simulink library "mssSimulink"  (R2024a)
settings: Solver=ode45  StartTime=0.0  StopTime=10.0  RelTol=1e-3
undefined symbols (not defined in the file): ABC, CN_data, CX_data, CY_data, D, G, Hoerner, K_supply, kt2ms, MA, magnitude, MRB, pathlength, RAO_Amp, RAO_Dir, RAO_Freq, RAO_Phase, RAO_Vel, RAO_yaw_back, RAO_yaw_quant, RAO_yaw_quantization_flag, rho_a, slcm, T_supply, table, vessel, vesselABC
libraries: $bdroot x99, simulink x13
(part 2 of 9)

== system mssSimulink/Marine craft models ==
  note: 3-DOF low-speed models
  note: 6-DOF low-speed models 6-DOF interface for 3-DOF models
  note: m-file models
  note: 4-DOF maneuveing models
  note: Nomoto models
  4-DOF naval vessel : Subsystem  mask(Naval Vessel Nonlinear Manoeuvring Model){x0=[kt2ms(15),0,0,0,0,0]'}
      mask prompts: x0 "Initial Condition x0=[u,v,p,r,phi,psi]"
      mask help:
      | Naval Vessel Model in 4 DOFs (surge,sway, roll, and yaw)
      | Input:
      | tau - vector of forces [X,Y,K,N]' in Newtons
      |
      | Output:
      | eta -  [phi,psi]'  Euler angles [rad]
      | nu  -  [u,v,p,r]   Linear and angular velocities in the body-fixed frame.
      |
      | Copyright 2005 NTNU
      | Author: Tristan Perez
      mask Help:
      | <p><font face="Arial">This is nonlinear manoeuvring model in 4 DOFs. This model
      | has been implemented usign the GNC vessel model block, and the </font>
      | <font face="Courier">m</font><font face="Arial"> file associated with the model
      | is </font></p>
      | <p><font face="Courier">MSS\VESSELS\navalvessel.m</font></p>
      | <p><font face="Arial">All the hydrodynamic data is in the above file.&nbsp; For
      | an example of use see&nbsp; the following demo:</font></p>
      | <p><font face="Courier">SIMULINK\DEMOS\demoNavalVesselMano.slxl</font></p>
      mask Display:
      | image(imread('simulink/figs/nvessel.jpg'))
      | color('white'); port_label('output', 1, 'eta')
      | color('white');port_label('output', 2, 'nu')
      | color('white'); port_label('input', 1, 'tau')
  6-DOF semisub : Subsystem  InitFcn=load MSS/VESSELS/models/rigModel/rig.mat  mask(6-DOF semisub){D=D, G=G, MA=MA, MRB=MRB}
      mask prompts: D "Linear damping matrix: D"; G "Spring matrix G:"; MA "System inertia added mass matrix: M"; MRB "System inertia rigid-body matrix"
      mask help:
      | Semisub low-speed model for DP.
      |
      | Inputs:
      |
      |    tau = 6 DOF control input vector (generalized force)
      |
      | Outputs:
      |
      |    eta = [x, y, z, phi, theta, psi]'
      |    nu  = [u, v, w, p, q, r]'
      mask Display:
      | image(imread('semisub.jpg'))
      | color('black'); port_label('output', 1, 'eta')
      | color('black'); port_label('output', 2, 'nu')
      | color('black'); port_label('input', 1, 'tau')
      | color('black'); port_label('input', 2, 'nu_c')
  6-DOF supply vessel interface : Subsystem
      mask Display: disp('6-DOF interface\n to 3-DOF vessel\n models')
  Container ship: L = 175 m : Subsystem  mask(m-file vessel model interface){vessmodel='container', dimu_model=2, dimx_model=10}
      mask prompts: vessmodel "m-file vessel model"; dimu_model "dim u"; dimx_model "dim x"
      mask help:
      | Simulink interface to the GNC toolbox m-file vessel models, type:
      |
      |    >help vesselmodels
      |
      | in the Matlab command window. A Simulink demo file is found under examples (demomf.mdl).
      |
      | Inputs/outputs:
      |
      |    u   = control input vector of dimension dimu
      |    xo = initial state vector of dimension dimx
      |    x   = state vector of dimension dimx
      mask Help:
      | Simulink interface to the GNC toolbox m-file vessel models.
      | Type >help vesselmodels in the Matlab command window to see a list of the m-file vessel models. The dimension of the state and input vectors are found  by typing >help "m-file"
      mask Display: disp('Integration of\n container.m\n\n x = [u v r x y psi p phi delta n]\n u = [delta_c n_c]')
  CyberShipII : Subsystem  LoadFcn=initCS2
      mask init:
      | D = [ 2.0000         0         0
      |          0    7.0000    0.1000
      |          0    0.1000    0.5000];
      | M = [  25.8000         0         0
      |          0   33.8000    1.0115
      |          0    1.0115    2.7600 ];
      mask Display:
      | image(imread('simulink/figs/cs.jpg'))
      | color('white'); port_label('output', 1, 'eta')
      | color('white');port_label('output', 2, 'nu')
      | color('white'); port_label('input', 1, 'tau')
  Deep submergence rescue vehicle (DSRV.m) : Subsystem
      mask Display: image('DSRV.jpg'); % Use "Edit Image" on toolstrip to change.
  Large tanker: L = 304 m : Subsystem  mask(m-file vessel model interface){vessmodel='tanker', dimu_model=3, dimx_model=8}
      mask prompts: vessmodel "m-file vessel model"; dimu_model "dim u"; dimx_model "dim x"
      mask help:
      | Simulink interface to the GNC toolbox m-file vessel models, type:
      |
      |    >help vesselmodels
      |
      | in the Matlab command window. A Simulink demo file is found under examples (demomf.mdl).
      |
      | Inputs/outputs:
      |
      |    u   = control input vector of dimension dimu
      |    xo = initial state vector of dimension dimx
      |    x   = state vector of dimension dimx
      mask Help:
      | Simulink interface to the GNC toolbox m-file vessel models.
      | Type >help vesselmodels in the Matlab command window to see a list of the m-file vessel models. The dimension of the state and input vectors are found  by typing >help "m-file"
      mask Display: disp('Integration of\n tanker.m\n\n x = [u v r x y psi delta n]\n u = [delta_c n_c h]')
  Mariner class cargo ship (2nd -order) : Subsystem  mask(Container ship (2nd-order model)){rate_max=5*(pi/180), delta_max=20*(pi/180), K=0.185, T1=118, T2=7.8, T3=18.5}
      mask prompts: rate_max "Max rudder rate: rate_max (rad/s)"; delta_max "Max rudder angle: delta_max (rad)"; K "Gain constant: K (1/s)"; T1 "Time constant: T1 (s)"; T2 "Time constant: T2 (s)"; T3 "Time constant: T3 (s)"
      mask Display:
      | image(imread('simulink/figs/mariner.jpg'))
      | color('white'); port_label('output', 1, 'psi')
      | color('white'); port_label('output', 2, 'r')
      | color('white'); port_label('output', 3, 'delta')
      | color('white'); port_label('input', 1, 'delta_c')
  Mariner class cargo ship (mariner.m) : Subsystem
      mask Display: image('mariner.jpg');
  Naval Postgraduate School AUV (npsAUV.m) : Subsystem
      mask Display: image('npsauv.png'); % Use "Edit Image" on toolstrip to change.
  Otter USV (otter.m) : Subsystem
      mask Display: image('otter.jpg'); % Use "Edit Image" on toolstrip to change.
  Remus 100 AUV (remus100.m) : Subsystem
      mask Display: image('remus100.jpg'); % Use "Edit Image" on toolstrip to change.
  Supply vessel : Subsystem  mask(Supply Vessel (surge, sway and yaw)){D=[5.0242e4 0 0; 0 2.7229e5 -4.3933e6; 0 -4.3933e6 4.1894e8], Minv=inv( [5.3122e6 0 0; 0 8.2831e6 0; 0 0 3.7454e9] )}
      mask prompts: D "Linear damping matrix: D"; Minv "Inverse inertia matrix: Minv"
      mask help:
      | DP model
      |
      | Inputs:
      |
      |    tau = 3 DOF control input vector (generalized force)
      |
      | Outputs:
      |
      |    eta = [x, y, psi]'
      |    nu  = [u, v, r]'
      mask Display:
      | image(imread('simulink/figs/supply.jpg'))
      | color('black'); port_label('output', 1, 'eta')
      | color('black'); port_label('output', 2, 'nu')
      | color('black'); port_label('input', 1, 'tau')
  Tanker (1st-order) : Subsystem  mask(Tanker (Nomoto 1st.-order)){rate_max=5*(pi/180), delta_max=20*(pi/180), K=-0.019, T=-153.7}
      mask prompts: rate_max "Max rudder rate: rate_max (rad/s):"; delta_max "Max rudder angle: delta_max  (rad)"; K "Gain constant: K (1/s)"; T "Time constant: T (s)"
      mask help:
      | Tanker: Nomoto 1st-order model
      |
      | Input:
      |
      |   delta_c = rudder angle command (rad)
      |
      | Outputs:
      |
      |    psi    = yaw angle (rad)
      |    r        = yaw rate (rad)
      |    delta = rudder angle from steering machine (rad)
      mask Display:
      | image(imread('simulink/figs/tanker.jpg'))
      | color('white'); port_label('output', 1, 'psi')
      | color('white'); port_label('output', 2, 'r')
      | color('white'); port_label('output', 3, 'delta')
      | color('white'); port_label('input', 1, 'delta_c')
  Tanker (2nd-order) : Subsystem  mask(Tanker (Nomoto 2nd-order model)){rate_max=5*(pi/180), delta_max=20*(pi/180), K=-0.019, T1=-124.1, T2=16.4, T3=46}
      mask prompts: rate_max "Max rudder rate: rate_max (rad/s)"; delta_max "Max rudder angle: delta_max (rad)"; K "Gain constant: K (1/s)"; T1 "Time constant: T1 (s)"; T2 "Time constant: T2 (s)"; T3 "Time constant: T3 (s)"
      mask help:
      | Tanker: Nomoto 2nd-order model
      |
      | Input:
      |
      |   delta_c = rudder angle command (rad)
      |
      | Outputs:
      |
      |    psi    = yaw angle (rad)
      |    r        = yaw rate (rad)
      |    delta = rudder angle from steering machine (rad)
      mask Display:
      | image(imread('simulink/figs/tanker.jpg'))
      | color('white'); port_label('output', 1, 'psi')
      | color('white'); port_label('output', 2, 'r')
      | color('white'); port_label('output', 3, 'delta')
      | color('white'); port_label('input', 1, 'delta_c')

== system mssSimulink/Modelling ==
  Control Surfaces : Subsystem
  Environmental Loads : Subsystem
  Hydromecanics : Subsystem
  Kinematics : Subsystem
  "Kinetics " : Subsystem
  Propulsion : Subsystem

== system mssSimulink/Navigation ==
  Estimators : Subsystem
  "Sensors " : Subsystem

== system mssSimulink/Utilities ==
  Dynamics : Subsystem
  Math Operations : Subsystem
  Simulation tools : Subsystem
  Visualization : Subsystem

== system mssSimulink/Control/Autopilots ==
  Course autopilot : Subsystem  mask{wn=1.2, zeta=1, T_nomoto=0.5, m=37.1}
      mask prompts: wn "Natural frequency: wn"; zeta "Relative damping ratio: zeta"; T_nomoto "Tme constant in yaw: T_nomoto"; m "Moment of inertia including added moment of inertia: Iz-Nrdot"
      mask help: PID pole-placement algorithm
      mask Display: disp('PID\n pole placement')
  "Course autopilot " : Subsystem  mask(Course Autopilot){T_nomoto=107.3, K_nomoto=0.185, Kp=1.45*0.9, Td=36, Ti=200}
      mask prompts: T_nomoto "Nomoto Time Constant: T"; K_nomoto "Nomoto gain: K"; Kp "Proportional Gain: Kp"; Td "Derivative Time: Td"; Ti "Integral Time: Ti"
      mask help: PID Autopilot with reference feedforward.
      mask Help: INPUTS: (1)  desired position, (2) desired velocity, (3) desired acceleration, (4) heading angle, (5) heading rate: OUTPUTS: (1) rudder angle
      mask Display: disp('PID\n tracking\n controller')
  Heading autopilot : Subsystem  mask(Course Autopilot){T_nomoto=1, K_nomoto=1, Kp=1, Td=0, Ti=0}
      mask prompts: T_nomoto "Nomoto Time Constant: T"; K_nomoto "Nomoto gain: K"; Kp "Proportional Gain: Kp"; Td "Derivative Time: Td"; Ti "Integral Time: Ti"
      mask help: PID Autopilot with reference feedforward.
      mask Help: INPUTS: (1)  desired position, (2) desired velocity, (3) desired acceleration, (4) heading angle, (5) heading rate: OUTPUTS: (1) rudder angle
      mask Display: disp('PID\n tracking\n controller')

== system mssSimulink/Control/DP ==
  Nonlinear PID : Subsystem  mask(Nonlinear DP Controller){Kp=diag([1 1 1]), Kd=diag([1 1 1]), Ki=diag([1 1 1])}
      mask prompts: Kp "Proportional Gain Matrix: Kp"; Kd "Derivative Gain Matrix: Kd"; Ki "Integral Gain Matrix: Ki"
      mask help: Nonlinear PID controller for Set-Point Reulation in Surge, Sway and Yaw
      mask Help:
      | The nonlinear  PID controller uses the rotation matrix in yaw for proper scaling of the surge, sway and yaw gains as a function of the yaw angle.
      | INPUTS: (1) eta_ref, (2) eta, (3) nu. OUPUTS: (1) tau.
      mask Display: disp('Nonlinear PID\n setpoint controller')

== system mssSimulink/Environment/Current ==
  North-East current : Subsystem

== system mssSimulink/Environment/Waves ==
  " Gaussian Random Process" : Subsystem  mask(Gaussian Random Process as a Sum of Sinusoids){areg=[], freq=[], phases=[]}
      mask prompts: areg "Vector of Amplitudes [A1;A2;...]:"; freq "Vector of frequencies [W1;W2;...]  [rad/sec]:"; phases "Vector of random phases [P1;P2;...]  [rad]:"
      mask help:
      | y = Sum_i  Ai *cos(w_i*t+ Phi_i)
      | Input:
      |  t --Simulation time from a clock block
      | Output:
      |  y--Realization of the random process y(t) (time series)
      | Dependency: None
      |
      | Copyright (C), NTNU  2004
      | Author: Tristan Perez
      mask Help: web(['file:///' which('Help_Gaussian_Random_Process.htm')]);
      mask Display:
      | plot([-ones(17,1)
      | 	0.6333
      |    -1.5315
      |    -0.5146
      |     0.5573
      |     1.2590
      |     1.8899
      |     1.5451
      |    -0.1055
      |    -1.0617
      |    -1.3645
      |    -1.3826
      |    -1.2742
      |     0.3850
      |     1.0225
      |     1.1108
      |     1.1270
      |     0.3762
      |    -0.6570
      |    -1.1216
      |    -0.2885
      |     0.9176
      |     0.7826
      |    -0.3229
      |    -1.2406
      |    -0.9331
      |    -0.2407
      |     0.4134
      |     0.8612
      |     0.3025
      |     0.2761
      |     0.3856
      |     0.3689
      |    -0.0188
      |     0.3654
      |    -0.4219
      |    -1.0260
      |    -1.3896
      |    -0.6530
      |     0.2512
      |     1.0351
      |     1.6496
      |     0.8313
      |    -1.2176
      |    -1.0937
      |     0.0268
      |     1.0361
      |     1.1728
      |    -0.2176
      |    -0.6390
      |    -1.1209
      |    -1.0516
      |    -0.4193
      |     0.7858
      |     0.8509
      |     0.4288
      |     0.0431
      |     0.0587
      |    -ones(15,1)])
      | port_label('input',1,'time')
      | port_label('output',1,'y')
  Encounter frequency correction : Subsystem  mask(Encounter frequency correction){}
      mask help:
      | This block transforms the frequencies and wave numbers in the Waves bus generated by the MSS Waves block to encounter frequencies and encounter wave numbers using the transformation:
      |
      | Omega_e = Omega - U*Omega^2*cos(Psi_r)/g
      |
      | where U is the vessel forward speed, Psi_r is the angle of the waves relative to the vessel.
      |
      | Inputs:
      | Waves - Bus of harmonic wave components generated by the MSS Waves block.
      | U          - Forward speed of the reference frame relative to NED (m/s) (Usually the low-frequency speed of the vessel)
      | Psi       - Yaw orientation of the reference frame relative to NED (rad) (Usually the low-frequency heading of the vessel)
      |
      | Outputs:
      | Waves - Bus of harmonic wave components with corrected wave frequencies and wave numbers.
      |
      | Copyright (C) 2005, NTNU
      | Author: Oyvind Notland Smogeli
  Linear 2nd-order wave spectrum : Subsystem  mask{sigma=1, w_0=1, lambda=0.1}
      mask prompts: sigma "Wave spectrum gain: sigma  (m)"; w_0 "Wave spectrum peak frequency: w_0  (rad/s)"; lambda "Rrelative damping ratio: lambda"
      mask init:
      | w = 0.01:0.1:3*w_0;
      mask Display:
      | plot(w,4*w_0*sigma^2.*w.^2./((w_0^2-w.^2).^2+4*(lambda*w_0.*w).^2))
      | port_label('input', 1, 'w')
      | port_label('output', 1, 'y')
  W_wave 2 W_enc (no absolute value) : Subsystem  mask(Wave frequency to Encounter Frequency){}
      mask help:
      | This block implements the transformation:
      |
      | We = W -U W^2 cos(Enc Aang) /g
      |
      | Inputs:
      | U---forward speed of the reference frame (m/sec) (sually the speed of the vessel)
      | W--vector of wave frequencies (rad/sec)
      | Enc. Angle-- (rad) convention: 0-following seas; pi/2-port beam seas; pi-head seas
      |
      | Outputs:
      | We--vector of encounter frequencies (rad/sec).
      | Ke-- vector of encounter wave numbers (Ke = We^2/g deep water assumption)
      | Copyright (C) 2005, NTNU
      | Author: Tristan Perez
      mask Help:
      | <p>This block implements the transformation: <br>
      | <br>
      | We = W -U W^2 cos(Enc Ang) /g <br>
      | <br>
      | Inputs:<br>
      | U---forward speed of the reference frame (m/sec) (Usually the speed of the
      | vessel)<br>
      | W--vector of wave frequencies (rad/sec)<br>
      | Enc. Angle-- (rad) convention: 0-following seas; pi/2-port beam seas; pi-head
      | seas<br>
      | <br>
      | Outputs:<br>
      | We--vector of encounter frequencies (rad/sec).<br>
      | Ke-- vector of encounter wave numbers (Ke = We^2/g deep water assumption)<br>
      | Copyright (C) 2005, NTNU<br>
      | Author: Tristan Perez </p>
  Wave velocitycalc : Subsystem  mask(Wave velocitycalc){}
      mask help: Caclulates the wave-induced water velocity in NED coordinates and surface elevation Zeta at the point [x y z] in NED. The Waves bus generated by the Waves module is needed as input.
  Waves : Subsystem  mask(Waves){spectrum_type=ITTC, disp_flag=on, plot_spectrum=off, plot_realization=off, hs=0.8, omega_peak=0, psi_mean=0, gamma=-1, spread=2, depth=inf, nfreq=20, ndir=10, energylim=0.005, freq_cutoff=3, dir_cutoff=0, rand_seed=123, rand_freq=on, rand_dir=on, Zeta_a=0, Omega=0, Phase=0, Wavenum=0, Psi=0}
      mask prompts: spectrum_type "Spectrum type"; disp_flag "Display initialization info in workspace window"; plot_spectrum "Plot spectrum"; plot_realization "Plot sea state realization (time-consuming)"; hs "Significant wave height Hs (m)"; omega_peak "Peak frequency omega_0 (rad/s)"; psi_mean "Mean wave direction (rad)"; gamma "Spectrum peakedness factor [1,7], 3.3 default, 0 for using DNV value"; spread "Wave spreading factor (1,2,3,4,5)"; depth "Average water depth (m), use inf for deep water"; nfreq "Number of frequencies in grid (recommended > 20)"; ndir "Number of directions in grid, 1 for long-crested waves"; energylim "Wave component energy limit [0 1] or number of waves (e.g. 50)"; freq_cutoff "Frequency cutoff factor [1.5, 5], default 3"; dir_cutoff "Direction cutoff [0, 3pi/8], default 0"; rand_seed "Random seed"; rand_freq "Random frequencies"; rand_dir "Random directions"; Zeta_a "Amplitude vector 'Zeta_a' (m)"; Omega "Frequency vector 'Omega' (rad/s)"; Phase "Phase vector 'Phase' (rad)"; Wavenum "Wavenumber vector 'Wavenum' (1/m)"; Psi "Direction vector 'Psi'  (rad)"
      mask help:
      | Calculate harmonic wave component parameters from a wave spectrum.
      | - Input one wave direction in the mask to get long-crested waves.
      | - Input zero peak frequency to get an expectation value from north sea statistical data.
      | - Input an integer > 1 for energylim to set the number of wave components fixed to nwaves = energylim.
      |
      | Copyright (C) 2004 NTNU
      | Author: Oyvind Notland Smogeli
      mask init:
      | if spectrum_type < 4
      | 	[Zeta_a, Omega, Phase, Wavenum, Psi] = Wave_init(spectrum_type, hs, omega_peak, psi_mean,...
      | 	gamma, spread, depth, nfreq, ndir, energylim, freq_cutoff, dir_cutoff, rand_freq, rand_dir,...
      | 	rand_seed, plot_spectrum, plot_realization, disp_flag);
      | end
      mask Help:
      | <font face="Arial">
      | <b>Project:</b> Marine Systems Simulator: MSS<br>
      | <br>
      | Define harmonic wave components describing the sea state by extracting
      | components from a given frequency and direction spectrum. The output from the
      | block is a bus containing the following wave parameter vectors:</font></p>
      | <p><font face="Arial"><b>Zeta_a</b>: Vector of harmonic wave amplitudes [m]<br>
      | <b>Omega: </b>Vector of harmonic wave frequencies [rad/s]<br>
      | <b>Phase: </b>Vector of harmonic wave phases (random) [rad]<br>
      | <b>Wavenum:</b> Vector of harmonic wave numbers [1/m]<br>
      | <b>Psi: </b>Vector of harmonic wave directions [rad]</font></p>
      | <p><font face="Arial">The time series of sea surface elevation Zeta(x,y,t) can
      | be obtained as</font></p>
      | <p><font face="Arial">Zeta(x,y,t) = Sum( Zeta_a(i)*cos(Omega(i)*t + Phase(i) - Wavenum(i)*(x*cos(Psi(i))
      | + y*sin(Psi(i)))) )</font></p>
      | <p><font face="Arial">where the sum is taken from i = 1 to i = n and n is the number of harmonic
      | wave components.</font></p>
      | <p>&nbsp;</p>
      | <p><font face="Arial">Input one wave direction to get long-crested waves.<br>
      | <br>
      | If the peak frequency is set to zero, then the peak frequency is obtained from
      | the sugnificant wave height usign a formula for the North Sea (Norsok):</font></p>
      | <p><font face="Arial">w0 = 2*pi/(4.883 + 2.68*Hs^0.54);</font></p>
      | 
      | <p>&nbsp;</p>
      | <p><font face="Arial">The energy limit (energylim) should be defined either as a positive factor
      | between 0 and 1, or as a positive integer. In the first case it will
      | discard all wave components with energy content less than this ratio of the
      | total energy content of the sea state. A recommended value is 0.005 or lower. In
      | the second case it will keep the nwaves = energylim most significant waves.</font></p>
      | <p>&nbsp;</p>
      | <p><font face="Arial">The wave elevation Zeta(x,y,t) at time t and at the coordinate (x,y) is found from the output vectors as:</font></p>
      | <p>&nbsp;</p>
      | <p><font face="Arial" color="#800000">References</font><ul>
      |   <li><font face="Arial">Sorensen, A.J. (2005) Lecture notes of TMR4240 &quot;Marine Cybernetics - Modelling and Control&quot;</font>
      |   <font face="Arial">Dept of Marine Technology NTNU.</font></li>
      |   <li><font face="Arial">Johannessen, K., T. S. Meling, S. Haver. Joint
      |   Distribution for Wind and<br>
      |   Waves in the Northern North Sea. IJOPE Vol. 12, No. 1, March 2002</font></li>
      |   <li>&nbsp;</li>
      |   </ul>
      | <p><font face="Arial">Johannessen, K., T. S. Meling, S. Haver. Joint
      | Distribution for Wind and<br>
      | Waves in the Northern North Sea. IJOPE Vol. 12, No. 1, March 2002</font><p>&nbsp;<p>
      |   <font face="Arial"><b>Author:</b> Oyvind Smogeli, September 2004 </font>
      | <p>&nbsp;</p>
      | <p>&nbsp;</p>
      mask TypeOptions spectrum_type: ITTC | Jonswap | Torsethaugen | Predefined waves
      mask Callback spectrum_type: Wave_callback;

== system mssSimulink/Environment/Wind ==
  Isherwood (1972) wind forces : Subsystem  mask(Isherwood wind forces){L=100, B=10, A_T=100, A_L=800, A_SS=200, S=130, C=30, M=0}
      mask prompts: L "L_oa: length overall (m)"; B "B: beam (m)"; A_T "A_T: transverse (xy-plane) projected area (m^2)"; A_L "A_L:  lateral (xz-plane) projected area (m^2)"; A_SS "A_SS: lateral projected area of superstructure (m^2)"; S "S: length of curve surrounding A_L minus A_wl  (exclude masts/ventilators)  (m)"; C "C: positive distance from bow to area center of A_L (m)"; M "M: number of distinct groups of masts or king posts seen in lateral projection"
      mask help:
      | Computation of the wind force/moment vector tau_wind in 6 DOF using the wind coeffisients of Isherwood (1972). The data file: Isherwood.m is loaded under initialization.
      |
      | Reference:
      |
      | R. M. Isherwood (1972). Wind Resistance of Merchant Ships. RINA Trans. Vol. 115, pp. 327-338.
      mask init:
      | eval('initIsherwood72')
      mask Help:
      | Computation of the wind force/moment vector tau_wind in 6 DOF using the wind coeffisients of Isherwood (1972). The data file: Isherwood.m is loaded under initialization.
      | 
      | Reference:
      | 
      | R. M. Isherwood (1972). Wind Resistance of Merchant Ships. RINA Trans. Vol. 115, pp. 327-338.
  Relative wind speed and angle of attack : Subsystem
  Wind : Subsystem  mask(Wind){page=1, Par_Wind_slowlyvar=off, Par_Wind_gust=off, Par_Wind_V=10, Par_Wind_angle=0, Par_Wind_spectrum_type=1, Par_Wind_z=10, Par_Wind_sample_time=0.1, Par_Wind_speed_T=10, Par_Wind_angle_T=10, Par_Wind_speed_noise_pow=1, Par_Wind_angle_noise_pow=0.01, Par_Wind_speed_rand_max=1, Par_Wind_angle_rand_max=pi/4, Par_Wind_speed_seed=123, Par_Wind_angle_seed=321, Par_Wind_phase_seed=1532, Par_Wind_kappa_H=0.0026, Par_Wind_L=1800, Par_Wind_minfreq=1E-4, Par_Wind_maxfreq=0.1, Par_Wind_nfreq=100}
      mask prompts: Par_Wind_slowlyvar "Include slowly-varing wind velocity and direction"; Par_Wind_gust "Include wind gust"; Par_Wind_V "Mean wind velocity [m/s]"; Par_Wind_angle "Mean wind angle [rad]"; Par_Wind_spectrum_type "Wind gust spectrum type"; Par_Wind_z "Height over water surface [m (for NORSOK wind spectrum)]"; Par_Wind_sample_time "Wind sample time [s]"; Par_Wind_speed_T "Wind speed time constant [s]"; Par_Wind_angle_T "Wind angle time constant [s]"; Par_Wind_speed_noise_pow "Wind speed noise power"; Par_Wind_angle_noise_pow "Wind angle noise power"; Par_Wind_speed_rand_max "Wind speed saturation [m/s] (max random variation about mean)"; Par_Wind_angle_rand_max "Wind angle saturation [rad] (max random variation about mean)"; Par_Wind_speed_seed "Wind speed random seed"; Par_Wind_angle_seed "Wind angle random seed"; Par_Wind_phase_seed "Wind gust phase seed"; Par_Wind_kappa_H "Sea surface drag coefficient for Harris wind spectrum (0.0026)"; Par_Wind_L "Scaling length for Harris wind spectrum (1800)"; Par_Wind_minfreq "Minimum frequency in gust [Hz] (1E-4)"; Par_Wind_maxfreq "Maximum frequency in gust [Hz] (0.1)"; Par_Wind_nfreq "Number of frequency components"
      mask help:
      | Generates wind speed and direction based on the mean angle and mean wind speed at 10 meters height. The total velocity is composed of a slowly-varying mean superposed with gusts based on a chosen wind spectrum. The direction is slowly-varying based on a random process.
      |
      | The wind spectrum types are:
      |
      | 1) Harris         (based on measurements over land)
      | 2) NORSOK   (based on measurements from the North Sea)
      mask Help:
      | <b>Part of the Marine Systems Simulator: MSS</b><p>Generate wind speed and direction based on the mean angle and mean wind
      | speed at 10 meters height. The total velocity is composed of a slowly-varying
      | mean superposed with gusts based on a chosen wind spectrum. The direction is
      | slowly-varying based on a random process.<br>
      | <br>
      | The wind spectrum types are:<br>
      | <br>
      | 1) Harris (based on measurements over land)<br>
      | 2) NORSOK (based on measurements from the North Sea)</p>
      | <p>The wind gust from the Harris spectrum is uniform over the height, whereas
      | the wind gust from the NORSOK spectrum varies with the height.</p>
      | <p>The random variation of the mean speed and angle can be limited by two saturation
      | parameters, which define the maximum random deviation from the mean value.<p><b>Outputs:
      | </b> </p>
      | <p>angle: [rad] Wind angle in the n-frame<br>
      | speed: [m/s] Wind velocity in the n-frame<p>
      | <b>Copyright NTNU 2005</b></p>
      | <p><b>Author:</b> Oyvind N. Smogeli, 2005-05-03</p>
      mask TypeOptions page: 1 | 2
      mask Callback page: MSS_mask_page(12);
      mask TypeOptions Par_Wind_spectrum_type: 1 | 2

== system mssSimulink/Guidance/LOS observer ==
  LOS command : Inport
  "         " : TransferFcn  Denominator=[1 0]
  Differentiator : TransferFcn  Numerator=[1/(alpha*K_f) 0]  Denominator="[1/(alpha*K_f)  1]"
  Observer gain : Gain  Gain=K_f  SaturateOnIntegerOverflow=on  OutDataTypeStr=Inherit: Same as input  ParamDataTypeStr=Inherit: Same as input
  Sum : Sum  Inputs=++|
  Sum2 : Sum  Inputs=|+-  InputSameDT=on  SaturateOnIntegerOverflow=on  OutDataTypeStr=Inherit: Same as first input
  ssa : $bdroot/Utilities/Math Operations/ssa  SystemSampleTime=-1  VariantActivationTime=update diagram  AllowFlexibleInterface=on  Latency=0  AutoFrameSizeCalculation=off
  LOSangle : Outport  InitialOutput=0  VectorParamsAs1DForOutWhenUnconnected=off
  LOSrate : Outport  Port=2  InitialOutput=0  VectorParamsAs1DForOutWhenUnconnected=off
  wires:
  LOS command/1 -> Sum2/1
  Sum2/1 -> ssa/1
  "         "/1 -> Sum2/2, Differentiator/1, LOSangle/1
  Observer gain/1 -> Sum/2
  ssa/1 -> Observer gain/1
  Sum/1 -> "         "/1
  Differentiator/1 -> LOSrate/1, Sum/1

== system mssSimulink/Guidance/Reference model ==
  desired position : Inport
  "    " : TransferFcn  Denominator=[1 0]
  "       " : Saturate  UpperLimit=v_max  LowerLimit=-v_max
  "         " : TransferFcn  Denominator=[1 0]
  Sum2 : Sum  Inputs=|+-  InputSameDT=on  SaturateOnIntegerOverflow=on  OutDataTypeStr=Inherit: Same as first input
  Sum5 : Sum  Inputs=|+-  InputSameDT=on  SaturateOnIntegerOverflow=on  OutDataTypeStr=Inherit: Same as first input
  damping : Gain  Gain=2*zeta_d*w_d  SaturateOnIntegerOverflow=on  OutDataTypeStr=Inherit: Same as input  ParamDataTypeStr=Inherit: Same as input
  low-pass filter : TransferFcn  Numerator=[w_d^3]  Denominator=[1 w_d]
  spring : Gain  Gain=w_d*w_d  SaturateOnIntegerOverflow=on  OutDataTypeStr=Inherit: Same as input  ParamDataTypeStr=Inherit: Same as input
  "desired position " : Outport  InitialOutput=0  VectorParamsAs1DForOutWhenUnconnected=off
  desired velocity : Outport  Port=2  InitialOutput=0  VectorParamsAs1DForOutWhenUnconnected=off
  desired acceleration : Outport  Port=3  InitialOutput=0  VectorParamsAs1DForOutWhenUnconnected=off
  wires:
  damping/1 -> Sum5/2
  "         "/1 -> "       "/1
  "    "/1 -> "desired position "/1, spring/1
  spring/1 -> Sum2/2
  Sum2/1 -> Sum5/1
  low-pass filter/1 -> Sum2/1
  desired position/1 -> low-pass filter/1
  Sum5/1 -> "         "/1, desired acceleration/1
  "       "/1 -> damping/1, "    "/1, desired velocity/1

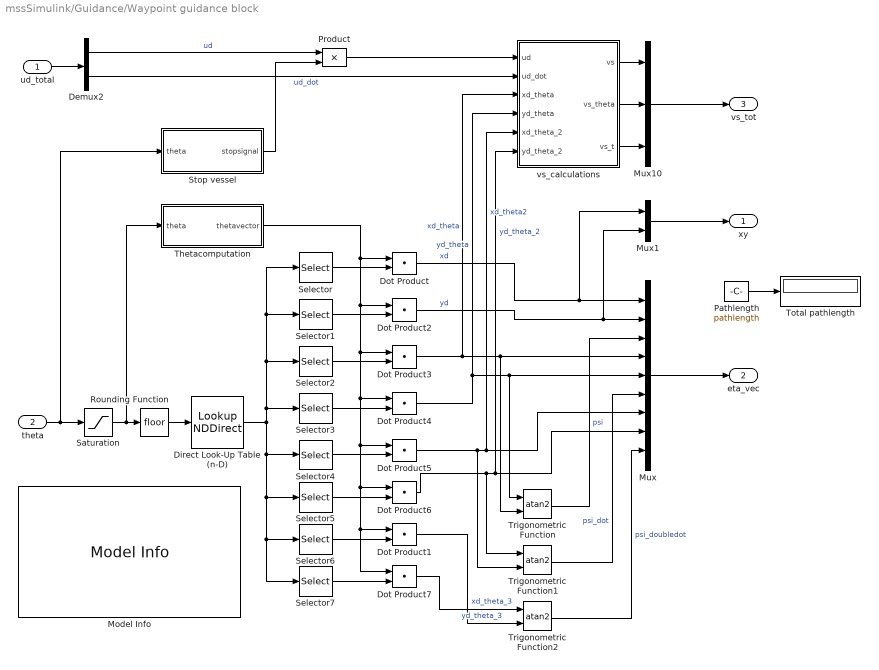
== system mssSimulink/Guidance/Waypoint guidance block ==
  ud_total : Inport  PortDimensions=2
  theta : Inport  Port=2
  Demux2 : Demux  Outputs=2
      settings: DisplayOption=none
  Direct Look-Up Table (n-D) : LookupNDDirect  InputsSelectThisObjectFromTable=Vector  Table=table  DiagnosticForOutOfRangeInput=None
  Dot Product{,1..7} (8 alike) : DotProduct  OutDataTypeStr=Inherit: Inherit via internal rule
  Model Info : simulink/Model-Wide Utilities/Model Info  Frame=on  DisplayStringWithTags=|  HorizontalTextAlignment=Center  LeftAlignmentValue=0.5
      | Guidance block.
      | Creates a three times differentiable path 
      | between the provided waypoints. The user 
      | can choose between cubic splines and a 
      | 5th order polynomial.
      | Author: Jorgen Corneliussen
      | Modified: %<ModifiedDate>
      | Version: %<ModelVersion>
  Mux : Mux  Inputs=9
  Mux1 : Mux  Inputs=2
  Mux10 : Mux  Inputs=3
  Pathlength : Constant  Value=pathlength
  Product : Product  SaturateOnIntegerOverflow=on  OutDataTypeStr=Inherit: Same as first input
  Rounding Function : Rounding
  Saturation : Saturate  UpperLimit=size(table,2) -0.001  LowerLimit=0
  Selector : Selector  InputPortWidth=size(table,1)  IndexOptions=Index vector (dialog)  Indices=[0*(size(table,1)/8)+1 :1*(size(table,1)/8)]  OutputSizes=1
  Selector1 : Selector  InputPortWidth=size(table,1)  IndexOptions=Index vector (dialog)  Indices=[1*(size(table,1)/8)+1 :2*(size(table,1)/8)]  OutputSizes=1
  Selector2 : Selector  InputPortWidth=size(table,1)  IndexOptions=Index vector (dialog)  Indices=[2*(size(table,1)/8)+1 :3*(size(table,1)/8)]  OutputSizes=1
  Selector3 : Selector  InputPortWidth=size(table,1)  IndexOptions=Index vector (dialog)  Indices=[3*(size(table,1)/8)+1 :4*(size(table,1)/8)]  OutputSizes=1
  Selector4 : Selector  InputPortWidth=size(table,1)  IndexOptions=Index vector (dialog)  Indices=[4*(size(table,1)/8)+1 :5*(size(table,1)/8)]  OutputSizes=1
  Selector5 : Selector  InputPortWidth=size(table,1)  IndexOptions=Index vector (dialog)  Indices=[5*(size(table,1)/8)+1 :6*(size(table,1)/8)]  OutputSizes=1
  Selector6 : Selector  InputPortWidth=size(table,1)  IndexOptions=Index vector (dialog)  Indices=[6*(size(table,1)/8)+1 :7*(size(table,1)/8)]  OutputSizes=1
  Selector7 : Selector  InputPortWidth=size(table,1)  IndexOptions=Index vector (dialog)  Indices=[7*(size(table,1)/8)+1 :8*(size(table,1)/8)]  OutputSizes=1
  Stop vessel : Subsystem
  Thetacomputation : Subsystem
  Total pathlength : Display
  Trigonometric Function : Trigonometry  Operator=atan2
  Trigonometric Function1 : Trigonometry  Operator=atan2
  Trigonometric Function2 : Trigonometry  Operator=atan2
  vs_calculations : Subsystem
  xy : Outport  VectorParamsAs1DForOutWhenUnconnected=off
  eta_vec : Outport  Port=2  VectorParamsAs1DForOutWhenUnconnected=off
  vs_tot : Outport  Port=3  VectorParamsAs1DForOutWhenUnconnected=off
  wires:
  theta/1 -> Saturation/1, Stop vessel/1(theta)
  ud_total/1 -> Demux2/1
  Thetacomputation/1(thetavector) -> Dot Product/1, Dot Product2/1, Dot Product4/1, Dot Product5/1, Dot Product6/1, Dot Product7/1, Dot Product1/1, Dot Product3/1
  Dot Product/1 -> Mux/1, Mux1/1  "xd"
  Dot Product2/1 -> Mux/2, Mux1/2  "yd"
  Mux/1 -> eta_vec/1
  Dot Product3/1 -> Trigonometric Function/2, Mux/4, vs_calculations/3(xd_theta)  "xd_theta"
  Dot Product4/1 -> Mux/5, Trigonometric Function/1, vs_calculations/4(yd_theta)  "yd_theta"
  Dot Product5/1 -> Trigonometric Function1/2, Mux/7, vs_calculations/5(xd_theta_2)  "xd_theta2"
  Dot Product6/1 -> Trigonometric Function1/1, Mux/8, vs_calculations/6(yd_theta_2)  "yd_theta_2"
  Dot Product1/1 -> Trigonometric Function2/2  "xd_theta_3"
  Dot Product7/1 -> Trigonometric Function2/1  "yd_theta_3"
  Trigonometric Function/1 -> Mux/3  "psi"
  Trigonometric Function1/1 -> Mux/6  "psi_dot"
  Trigonometric Function2/1 -> Mux/9  "psi_doubledot"
  Mux10/1 -> vs_tot/1
  vs_calculations/1(vs) -> Mux10/1
  vs_calculations/3(vs_t) -> Mux10/3
  vs_calculations/2(vs_theta) -> Mux10/2
  Saturation/1 -> Rounding Function/1, Thetacomputation/1(theta)
  Selector/1 -> Dot Product/2
  Selector1/1 -> Dot Product2/2
  Selector2/1 -> Dot Product3/2
  Selector3/1 -> Dot Product4/2
  Selector4/1 -> Dot Product5/2
  Selector5/1 -> Dot Product6/2
  Selector6/1 -> Dot Product1/2
  Selector7/1 -> Dot Product7/2
  Direct Look-Up Table (n-D)/1 -> Selector/1, Selector1/1, Selector2/1, Selector3/1, Selector4/1, Selector5/1, Selector7/1, Selector6/1
  Rounding Function/1 -> Direct Look-Up Table (n-D)/1
  Demux2/1 -> Product/1  "ud"
  Product/1 -> vs_calculations/1(ud)
  Stop vessel/1(stopsignal) -> Product/2
  Demux2/2 -> vs_calculations/2(ud_dot)  "ud_dot"
  Mux1/1 -> xy/1
  Pathlength/1 -> Total pathlength/1

== system mssSimulink/Guidance/Zigzag test rudder command  ==
  Rudder Ang : Inport
  "Yaw Ang  " : Inport  Port=2
  Matrix Gain4 : Gain  Gain=[-1]  Multiplication=Matrix(K*u)  SaturateOnIntegerOverflow=on  OutDataTypeStr=Inherit: Same as input  ParamDataTypeStr=Inherit: Same as input
  Sum3 : Sum  InputSameDT=on  SaturateOnIntegerOverflow=on  OutDataTypeStr=Inherit: Same as first input
  Switch : Switch
  test signal4 : Step  Time=0  After=RL  SampleTime=0
  "Rudder Command " : Outport  VectorParamsAs1DForOutWhenUnconnected=off
  wires:
  test signal4/1 -> Switch/1, Matrix Gain4/1
  Matrix Gain4/1 -> Switch/3
  Sum3/1 -> Switch/2
  Rudder Ang/1 -> Sum3/1
  "Yaw Ang  "/1 -> Sum3/2
  Switch/1 -> "Rudder Command "/1

== system mssSimulink/Hydrodynamics/6-DOF DP model (zero-speed model with fluid memory) ==
  tau_wave : Inport
  tau : Inport  Port=2
  v_c^n : Inport  Port=3
  6- DOF transformation : $bdroot/Modelling/Kinematics/6 DOF transformation  SystemSampleTime=-1  VariantActivationTime=update diagram  AllowFlexibleInterface=on  Latency=0  AutoFrameSizeCalculation=off
  B(inf) * nu_r + Bv(0) * nu_r : Product  Multiplication=Matrix(*)  SaturateOnIntegerOverflow=on  OutDataTypeStr=Inherit: Same as first input
  B(inf) + Bv(0) : Constant  Value=vessel.B(:,:,end) + vessel.Bv(:,:,1)
  "Cross-flow drag and surge resistance " : $bdroot/Hydrodynamics/Cross-flow drag and surge resistance  N=20  Lpp=vessel.main.Lpp  CD=CY_2D  Cx=CX  Ax=Axc  Ay=Ayc  rho_w=rho
  "Fluid memory effetcs " : $bdroot/Hydrodynamics/Fluid memory effetcs  SystemSampleTime=-1  VariantActivationTime=update diagram  AllowFlexibleInterface=on  Latency=0  AutoFrameSizeCalculation=off
  G*eta : Product  Multiplication=Matrix(*)  SaturateOnIntegerOverflow=on  OutDataTypeStr=Inherit: Same as first input
  "Integrator1 " : Integrator
  Integrator2 : Integrator
  Invers inertia matrix : Constant  Value=ABC.Minv
  Minv*tau : Product  Inputs=**  Multiplication=Matrix(*)  SaturateOnIntegerOverflow=on  OutDataTypeStr=Inherit: Same as first input
  Mux : Mux  Inputs=6
  Mux1 : Mux  Inputs=2
  Selector : Selector  InputPortWidth=6  IndexOptions=Index vector (dialog)  Indices=[6]  OutputSizes=1
  Spring stiffness : Constant  Value=ABC.G
  Sum : Sum  Inputs=|+-  SaturateOnIntegerOverflow=on
  Sum1 : Sum  Inputs=|+-  SaturateOnIntegerOverflow=on
  Sum2 : Sum  Inputs=|+-  SaturateOnIntegerOverflow=on
  Sum3 : Sum  Inputs=|++  SaturateOnIntegerOverflow=on
  Sum5 : Sum  Inputs=|++  SaturateOnIntegerOverflow=on
  Sum6 : Sum  Inputs=-+|  SaturateOnIntegerOverflow=on
  "Transposed rotation matrix in yaw " : $bdroot/Modelling/Kinematics/Transposed rotation  matrix in yaw
  zero : Constant  Value=0
  "zero  " : Constant  Value=[0 0 0]'
  eta : Outport
  nu : Outport  Port=2
  wires:
  Sum5/1 -> Sum2/1
  "Fluid memory effetcs "/1 -> Sum/2
  Sum3/1 -> Sum5/1
  tau_wave/1 -> Sum3/2
  tau/1 -> Sum1/1
  G*eta/1 -> Sum1/2
  Integrator2/1 -> 6- DOF transformation/1, Selector/1, eta/1, G*eta/2
  6- DOF transformation/1 -> Integrator2/1
  Minv*tau/1 -> "Integrator1 "/1
  Invers inertia matrix/1 -> Minv*tau/1
  Spring stiffness/1 -> G*eta/1
  Sum1/1 -> Sum3/1
  Sum/1 -> Minv*tau/2
  "Integrator1 "/1 -> 6- DOF transformation/2, nu/1, Sum6/2  "nu"
  "Cross-flow drag and surge resistance "/1 -> Mux/1
  "Cross-flow drag and surge resistance "/2 -> Mux/2
  "Cross-flow drag and surge resistance "/3 -> Mux/6
  zero/1 -> Mux/4, Mux/3, Mux/5
  Mux/1 -> Sum5/2
  v_c^n/1 -> "Transposed rotation matrix in yaw "/2
  Sum6/1 -> "Fluid memory effetcs "/1, "Cross-flow drag and surge resistance "/1, B(inf) * nu_r + Bv(0) * nu_r/2  "nu_r"
  B(inf) + Bv(0)/1 -> B(inf) * nu_r + Bv(0) * nu_r/1
  Sum2/1 -> Sum/1
  B(inf) * nu_r + Bv(0) * nu_r/1 -> Sum2/2
  Selector/1 -> "Transposed rotation matrix in yaw "/1
  "Transposed rotation matrix in yaw "/1 -> Mux1/1  "v_c^b"
  "zero  "/1 -> Mux1/2
  Mux1/1 -> Sum6/1  "nu_c"

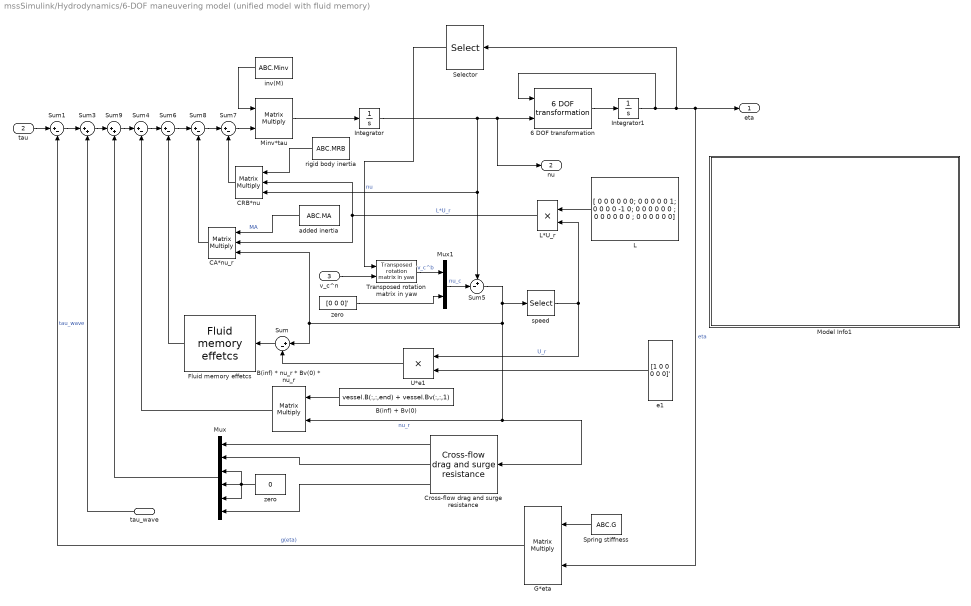
== system mssSimulink/Hydrodynamics/6-DOF maneuvering model (unified model with fluid memory) ==
  tau_wave : Inport
  tau : Inport  Port=2
  v_c^n : Inport  Port=3
  "6 DOF transformation " : $bdroot/Modelling/Kinematics/6 DOF transformation  SystemSampleTime=-1  VariantActivationTime=update diagram  AllowFlexibleInterface=on  Latency=0  AutoFrameSizeCalculation=off
  B(inf) * nu_r * Bv(0) * nu_r : Product  Multiplication=Matrix(*)  SaturateOnIntegerOverflow=on  OutDataTypeStr=Inherit: Same as first input
  B(inf) + Bv(0) : Constant  Value=vessel.B(:,:,end) + vessel.Bv(:,:,1)
  CA*nu_r : Product  Inputs=3  Multiplication=Matrix(*)  RndMeth=Zero
  CRB*nu : Product  Inputs=3  Multiplication=Matrix(*)  RndMeth=Zero
  "Cross-flow drag and surge resistance " : $bdroot/Hydrodynamics/Cross-flow drag and surge resistance  N=20  Lpp=vessel.main.Lpp  CD=CY_2D  Cx=CX  Ax=Axc  Ay=Ayc  rho_w=rho
  "Fluid memory effetcs " : $bdroot/Hydrodynamics/Fluid memory effetcs  SystemSampleTime=-1  VariantActivationTime=update diagram  AllowFlexibleInterface=on  Latency=0  AutoFrameSizeCalculation=off
  G*eta : Product  Multiplication=Matrix(*)  SaturateOnIntegerOverflow=on  OutDataTypeStr=Inherit: Same as first input
  Integrator : Integrator
  Integrator1 : Integrator
  L : Constant  Value=|
      | [ 0     0     0     0     0     0;   0     0     0     0     0     1;
      |      0     0     0     0    -1     0;	
      |      0     0     0     0     0     0	;
      |      0     0     0     0     0     0	
      | ;     0     0     0     0     0     0]
  L*U_r : Product  RndMeth=Zero
  Minv*tau : Product  Inputs=**  Multiplication=Matrix(*)  SaturateOnIntegerOverflow=on  OutDataTypeStr=Inherit: Same as first input
  Model Info1 : Subsystem  LoadFcn=slcm LoadBlock;  InitFcn=slcm('UpdateAllCMBlocksInThisModelInit')  mask(CMBlock){InitialSaveTempField=, InitialBlockCM=None, BlockCM=None, Frame=on, SaveTempField=, DisplayStringWithTags=|, MaskDisplayString=This is an example block based on Perez and Fossen (2007).\nThe model includes speed-dependent fluid memory effects \ncross-flow drag and surge resistance (quadratic drag).\nYou must inlcude maneuvering coefficients your self. \n\nAlso notice that viscous roll damping is computed under the assumption \nof zero speed. Forward speed effects can, however, be added if necessary.\n\nReference\nT. Perez and T. I. Fossen (2007). Kinematic Models for Seakeeping\nand Maneuvering of Marine Vessels. Modeling, Identification\nand Control, MIC-28(1):1-12.\n\nDownload link: www.marinecontrol.org\n\nAuthor: Thor I. Fossen\nSat Jun 08 08:27:48 2024, HorizontalTextAlignment=Left, LeftAlignmentValue=0.02, SourceBlockDiagram=marine_hydro, TagMaxNumber=20, CMTag1=, CMTag2=, CMTag3=, CMTag4=, CMTag5=, CMTag6=, CMTag7=, CMTag8=, CMTag9=, CMTag10=, CMTag11=, CMTag12=, CMTag13=, CMTag14=, CMTag15=, CMTag16=, CMTag17=, CMTag18=, CMTag19=, CMTag20=}
      mask DisplayStringWithTags=|
      | This is an example block based on Perez and Fossen (2007).\nThe model includes speed-dependent fluid memory effects
      | cross-flow drag and surge resistance (quadratic drag).\nYou must inlcude maneuvering coefficients your self. \n
      | Also notice that viscous roll damping is computed under the assumption \nof zero speed. Forward speed effects can, however, be added if necessary.
      |
      | Reference
      | T. Perez and T. I. Fossen (2007). Kinematic Models for Seakeeping
      | and Maneuvering of Marine Vessels. Modeling, Identification\nand Control, MIC-28(1):1-12.\n
      | Download link: www.marinecontrol.org
      |
      | Author: Thor I. Fossen
      | %<LastModificationDate>
      mask help: This block allows revision control information to be displayed within the model.
      settings: CopyFcn=slcm CopyBlock;  DeleteFcn=slcm Cancel;  PostSaveFcn=slcm('UpdateAllCMBlocksInThisModel')  NameChangeFcn=slcm Rename;  OpenFcn=slcm
      mask Display: text(str2num(LeftAlignmentValue), 0.5, MaskDisplayString, 'HorizontalAlignment', HorizontalTextAlignment)
  Mux : Mux  Inputs=6
  Mux1 : Mux  Inputs=2
  Selector : Selector  InputPortWidth=6  IndexOptions=Index vector (dialog)  Indices=[6]  OutputSizes=1
  Spring stiffness : Constant  Value=ABC.G
  Sum : Sum  Inputs=|+-
  Sum{1,4,6..8} (5 alike) : Sum  Inputs=|+-  SaturateOnIntegerOverflow=on
  Sum3 : Sum  Inputs=|++  SaturateOnIntegerOverflow=on
  Sum5 : Sum  Inputs=+-|  SaturateOnIntegerOverflow=on
  Sum9 : Sum  Inputs=|++  SaturateOnIntegerOverflow=on
  "Transposed rotation matrix in yaw " : $bdroot/Modelling/Kinematics/Transposed rotation  matrix in yaw
  U*e1 : Product  RndMeth=Zero
  added inertia : Constant  Value=ABC.MA
  e1 : Constant  Value=[1 0 0 0 0 0]'  VectorParams1D=off
  inv(M) : Constant  Value=ABC.Minv
  rigid body inertia : Constant  Value=ABC.MRB
  speed : Selector  InputPortWidth=6  IndexOptions=Index vector (dialog)  Indices=[1]  OutputSizes=1
  zero : Constant  Value=0
  "zero  " : Constant  Value=[0 0 0]'
  eta : Outport
  nu : Outport  Port=2
  wires:
  Minv*tau/1 -> Integrator/1
  Sum4/1 -> Sum6/1
  Sum6/1 -> Sum8/1
  Sum3/1 -> Sum9/1
  tau_wave/1 -> Sum3/2  "tau_wave"
  tau/1 -> Sum1/1
  rigid body inertia/1 -> CRB*nu/1
  G*eta/1 -> Sum1/2  "g(eta)"
  Integrator1/1 -> Selector/1, eta/1, G*eta/2, "6 DOF transformation "/1  "eta"
  "6 DOF transformation "/1 -> Integrator1/1
  added inertia/1 -> CA*nu_r/1  "MA"
  Spring stiffness/1 -> G*eta/1
  Sum1/1 -> Sum3/1
  Integrator/1 -> "6 DOF transformation "/2, nu/1, CRB*nu/3, Sum5/1  "nu"
  B(inf) + Bv(0)/1 -> B(inf) * nu_r * Bv(0) * nu_r/1
  B(inf) * nu_r * Bv(0) * nu_r/1 -> Sum4/2
  v_c^n/1 -> "Transposed rotation matrix in yaw "/2
  Sum5/1 -> CA*nu_r/3, Sum/1, B(inf) * nu_r * Bv(0) * nu_r/2, "Cross-flow drag and surge resistance "/1, speed/1  "nu_r"
  Sum7/1 -> Minv*tau/2
  "Fluid memory effetcs "/1 -> Sum6/2
  CRB*nu/1 -> Sum7/2
  Sum8/1 -> Sum7/1
  CA*nu_r/1 -> Sum8/2
  "Cross-flow drag and surge resistance "/1 -> Mux/1
  "Cross-flow drag and surge resistance "/2 -> Mux/2
  "Cross-flow drag and surge resistance "/3 -> Mux/6
  zero/1 -> Mux/4, Mux/3, Mux/5
  Sum9/1 -> Sum4/1
  Mux/1 -> Sum9/2
  L/1 -> L*U_r/1
  L*U_r/1 -> CRB*nu/2, CA*nu_r/2  "L*U_r"
  Sum/1 -> "Fluid memory effetcs "/1
  U*e1/1 -> Sum/2
  e1/1 -> U*e1/2
  inv(M)/1 -> Minv*tau/1
  speed/1 -> U*e1/1, L*U_r/2  "U_r"
  Selector/1 -> "Transposed rotation matrix in yaw "/1
  "Transposed rotation matrix in yaw "/1 -> Mux1/1  "v_c^b"
  Mux1/1 -> Sum5/2  "nu_c"
  "zero  "/1 -> Mux1/2

== system mssSimulink/Hydrodynamics/Cross-flow drag and surge resistance ==
  nu_r : Inport
  "2D drag coefficient " : Constant  Value=CD
  Abs1 : Abs
  Cross-flow drag trapezoidal integration : Subsystem  TreatAsAtomicUnit=on
  Drag coefficient : Constant  Value=Cx
  Frontal area : Constant  Value=Ax
  Gain : Gain  Gain=-0.5  SaturateOnIntegerOverflow=on  OutDataTypeStr=Inherit: Same as input  ParamDataTypeStr=Inherit: Same as input
  Gain1 : Gain  Gain=-0.5  SaturateOnIntegerOverflow=on  OutDataTypeStr=Inherit: Same as input  ParamDataTypeStr=Inherit: Same as input
  Gain2 : Gain  Gain=0.5  SaturateOnIntegerOverflow=on  OutDataTypeStr=Inherit: Same as input  ParamDataTypeStr=Inherit: Same as input
  Gain3 : Gain  Gain=-1  SaturateOnIntegerOverflow=on  OutDataTypeStr=Inherit: Same as input  ParamDataTypeStr=Inherit: Same as input
  Lpp : Constant  Value=Lpp
  N : Constant  Value=N
  Product5 : Product  Inputs=3  SaturateOnIntegerOverflow=on  OutDataTypeStr=Inherit: Same as first input
  Product7 : Product  SaturateOnIntegerOverflow=on  OutDataTypeStr=Inherit: Same as first input
  Product8 : Product  SaturateOnIntegerOverflow=on  OutDataTypeStr=Inherit: Same as first input
  Selector : Selector  InputPortWidth=6  IndexOptions=Index vector (dialog)  Indices=[2]  OutputSizes=1
  Selector1 : Selector  InputPortWidth=6  IndexOptions=Index vector (dialog)  Indices=[6]  OutputSizes=1
  Selector2 : Selector  InputPortWidth=6  IndexOptions=Index vector (dialog)  Indices=[1]  OutputSizes=1
  Sum : Sum  Inputs=+-|  InputSameDT=on  SaturateOnIntegerOverflow=on  OutDataTypeStr=Inherit: Same as first input
  Transversal area/Lpp : Constant  Value=Ay/Lpp
  constant : Constant
  dx : Product  Inputs=/*  RndMeth=Zero
  dx1 : Product  Inputs=4  RndMeth=Zero
  dx2 : Product  Inputs=4  RndMeth=Zero
  rho : Constant  Value=rho_w
  X_drag : Outport
  Y_drag : Outport  Port=2
  N_drag : Outport  Port=3
  wires:
  Drag coefficient/1 -> Product5/2
  rho/1 -> Product5/3, dx2/2, dx1/2
  dx2/1 -> N_drag/1
  Gain/1 -> dx2/1
  dx1/1 -> Y_drag/1
  Gain1/1 -> dx1/1
  nu_r/1 -> Selector1/1, Selector/1, Selector2/1
  Product8/1 -> Gain3/1
  Gain3/1 -> X_drag/1
  Cross-flow drag trapezoidal integration/1(sum1) -> Gain1/1
  Cross-flow drag trapezoidal integration/2(sum2) -> Gain/1
  Selector/1 -> Cross-flow drag trapezoidal integration/3(v_r)  "v_r"
  Selector1/1 -> Cross-flow drag trapezoidal integration/4(r)  "r"
  Lpp/1 -> dx/2
  constant/1 -> Sum/2
  dx/1 -> Cross-flow drag trapezoidal integration/2(dx)
  Sum/1 -> dx/1  "N-1"
  N/1 -> Cross-flow drag trapezoidal integration/1(N), Sum/1  "N"
  Transversal area/Lpp/1 -> dx1/3, dx2/3
  "2D drag coefficient "/1 -> dx1/4, dx2/4
  Gain2/1 -> Product5/1
  Frontal area/1 -> Gain2/1
  Selector2/1 -> Product7/2, Abs1/1  "u_r"
  Abs1/1 -> Product7/1
  Product7/1 -> Product8/1
  Product5/1 -> Product8/2

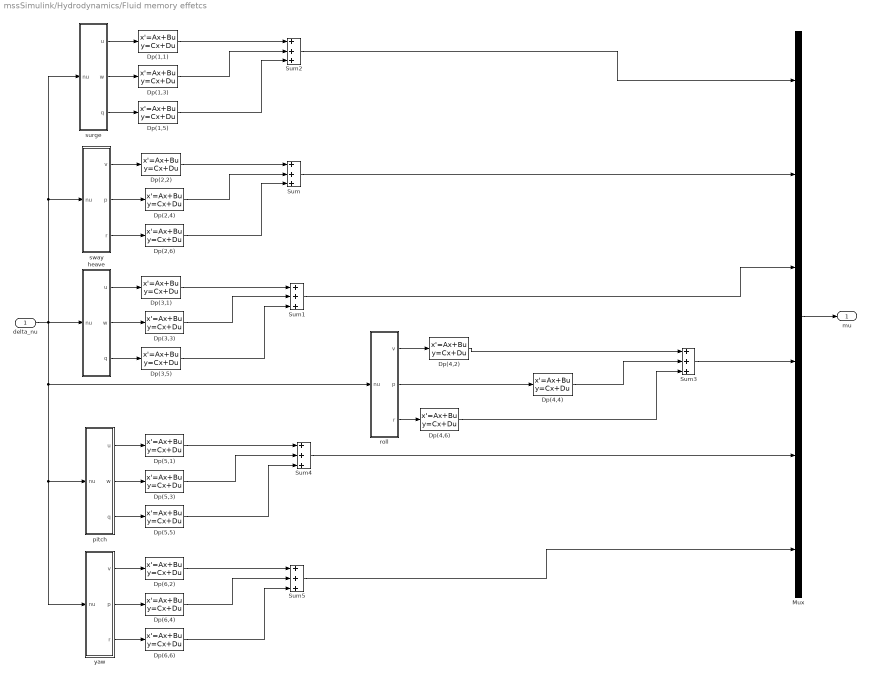
== system mssSimulink/Hydrodynamics/Fluid memory effetcs ==
  delta_nu : Inport
  Dp(1,1) : StateSpace  A=ABC.Ar{1,1}  B=ABC.Br{1,1}  C=ABC.Cr{1,1}  D=ABC.Dr{1,1}  InitialCondition=0
  Dp(1,3) : StateSpace  A=ABC.Ar{1,3}  B=ABC.Br{1,3}  C=ABC.Cr{1,3}  D=ABC.Dr{1,3}  InitialCondition=0
  Dp(1,5) : StateSpace  A=ABC.Ar{1,5}  B=ABC.Br{1,5}  C=ABC.Cr{1,5}  D=ABC.Dr{1,5}  InitialCondition=0
  Dp(2,2) : StateSpace  A=ABC.Ar{2,2}  B=ABC.Br{2,2}  C=ABC.Cr{2,2}  D=ABC.Dr{2,2}  InitialCondition=0
  Dp(2,4) : StateSpace  A=ABC.Ar{2,4}  B=ABC.Br{2,4}  C=ABC.Cr{2,4}  D=ABC.Dr{2,4}  InitialCondition=0
  Dp(2,6) : StateSpace  A=ABC.Ar{2,6}  B=ABC.Br{2,6}  C=ABC.Cr{2,6}  D=ABC.Dr{2,6}  InitialCondition=0
  Dp(3,1) : StateSpace  A=ABC.Ar{3,1}  B=ABC.Br{3,1}  C=ABC.Cr{3,1}  D=ABC.Dr{3,1}  InitialCondition=0
  Dp(3,3) : StateSpace  A=ABC.Ar{3,3}  B=ABC.Br{3,3}  C=ABC.Cr{3,3}  D=ABC.Dr{3,3}  InitialCondition=0
  Dp(3,5) : StateSpace  A=ABC.Ar{3,5}  B=ABC.Br{3,5}  C=ABC.Cr{3,5}  D=ABC.Dr{3,5}  InitialCondition=0
  Dp(4,2) : StateSpace  A=ABC.Ar{4,2}  B=ABC.Br{4,2}  C=ABC.Cr{4,2}  D=ABC.Dr{4,2}  InitialCondition=0
  Dp(4,4) : StateSpace  A=ABC.Ar{4,4}  B=ABC.Br{4,4}  C=ABC.Cr{4,4}  D=ABC.Dr{4,4}  InitialCondition=0
  Dp(4,6) : StateSpace  A=ABC.Ar{4,6}  B=ABC.Br{4,6}  C=ABC.Cr{4,6}  D=ABC.Dr{4,6}  InitialCondition=0
  Dp(5,1) : StateSpace  A=ABC.Ar{5,1}  B=ABC.Br{5,1}  C=ABC.Cr{5,1}  D=ABC.Dr{5,1}  InitialCondition=0
  Dp(5,3) : StateSpace  A=ABC.Ar{5,3}  B=ABC.Br{5,3}  C=ABC.Cr{5,3}  D=ABC.Dr{5,3}  InitialCondition=0
  Dp(5,5) : StateSpace  A=ABC.Ar{5,5}  B=ABC.Br{5,5}  C=ABC.Cr{5,5}  D=ABC.Dr{5,5}  InitialCondition=0
  Dp(6,2) : StateSpace  A=ABC.Ar{6,2}  B=ABC.Br{6,2}  C=ABC.Cr{6,2}  D=ABC.Dr{6,2}  InitialCondition=0
  Dp(6,4) : StateSpace  A=ABC.Ar{6,4}  B=ABC.Br{6,4}  C=ABC.Cr{6,4}  D=ABC.Dr{6,4}  InitialCondition=0
  Dp(6,6) : StateSpace  A=ABC.Ar{6,6}  B=ABC.Br{6,6}  C=ABC.Cr{6,6}  D=ABC.Dr{6,6}  InitialCondition=0
  Mux : Mux  Inputs=6
  Sum{,1..5} (6 alike) : Sum  Inputs=+++  SaturateOnIntegerOverflow=on
  heave : Subsystem
  pitch : Subsystem
  roll : Subsystem
  surge : Subsystem
  sway : Subsystem
  yaw : Subsystem
  mu : Outport
  wires:
  Sum4/1 -> Mux/5
  Dp(2,2)/1 -> Sum/1
  Dp(2,4)/1 -> Sum/2
  Dp(2,6)/1 -> Sum/3
  Sum/1 -> Mux/2
  sway/1(v) -> Dp(2,2)/1
  sway/2(p) -> Dp(2,4)/1
  sway/3(r) -> Dp(2,6)/1
  Dp(3,3)/1 -> Sum1/2
  Dp(3,5)/1 -> Sum1/3
  Sum1/1 -> Mux/3
  heave/3(q) -> Dp(3,5)/1
  heave/2(w) -> Dp(3,3)/1
  heave/1(u) -> Dp(3,1)/1
  Dp(3,1)/1 -> Sum1/1
  delta_nu/1 -> heave/1(nu), sway/1(nu), surge/1(nu), roll/1(nu), pitch/1(nu), yaw/1(nu)
  Mux/1 -> mu/1
  Dp(1,3)/1 -> Sum2/2
  Dp(1,5)/1 -> Sum2/3
  Sum2/1 -> Mux/1
  surge/3(q) -> Dp(1,5)/1
  surge/2(w) -> Dp(1,3)/1
  surge/1(u) -> Dp(1,1)/1
  Dp(1,1)/1 -> Sum2/1
  Dp(4,2)/1 -> Sum3/1
  Dp(4,6)/1 -> Sum3/3
  roll/1(v) -> Dp(4,2)/1
  roll/3(r) -> Dp(4,6)/1
  Dp(5,3)/1 -> Sum4/2
  Dp(5,5)/1 -> Sum4/3
  pitch/3(q) -> Dp(5,5)/1
  pitch/2(w) -> Dp(5,3)/1
  pitch/1(u) -> Dp(5,1)/1
  Dp(5,1)/1 -> Sum4/1
  Sum3/1 -> Mux/4
  Dp(6,2)/1 -> Sum5/1
  Dp(6,4)/1 -> Sum5/2
  Dp(6,6)/1 -> Sum5/3
  yaw/1(v) -> Dp(6,2)/1
  yaw/2(p) -> Dp(6,4)/1
  yaw/3(r) -> Dp(6,6)/1
  Sum5/1 -> Mux/6
  roll/2(p) -> Dp(4,4)/1
  Dp(4,4)/1 -> Sum3/2
